simulink model "joystick_setup"  (R2018b)
settings: Solver=VariableStepAuto  StartTime=0.0  StopTime=30  RelTol=1e-3
libraries: joystick_lib x2, matlabinput_lib x1, aerolibanimutils x1
settings Model: Creator=Yannic  LastModifiedBy=jonas
settings DataIOCC: SaveOutput=off  SaveTime=off

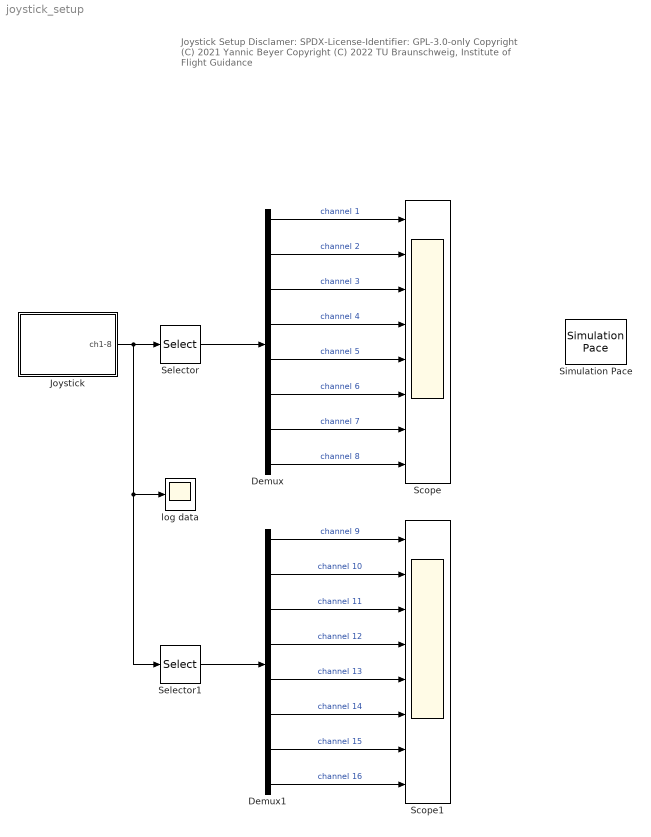
== system joystick_setup ==
  note: Joystick Setup
      |
      | Disclamer:
      | SPDX-License-Identifier: GPL-3.0-only
      |
      | Copyright (C) 2021 Yannic Beyer
      | Copyright (C) 2022 TU Braunschweig, Institute of Flight Guidance
  Demux : Demux  Outputs=8
  Demux1 : Demux  Outputs=8
  Joystick : Subsystem
  Scope : Scope  NumInputPorts=8
  Scope1 : Scope  NumInputPorts=8
  Selector : Selector  InputPortWidth=16  IndexOptions=Index vector (dialog)  Indices=1:8  OutputSizes=1
  Selector1 : Selector  InputPortWidth=16  IndexOptions=Index vector (dialog)  Indices=9:16  OutputSizes=1
  Simulation Pace : aerolibanimutils/Simulation Pace  SimulationPace=1  SleepMode=Auto  OutputPaceError=off  SampleTime=1/30
  log data : Scope
  wires:
  Demux/1 -> Scope/1  "channel 1"
  Demux/2 -> Scope/2  "channel 2"
  Demux/3 -> Scope/3  "channel 3"
  Demux/4 -> Scope/4  "channel 4"
  Demux/5 -> Scope/5  "channel 5"
  Demux/6 -> Scope/6  "channel 6"
  Demux/7 -> Scope/7  "channel 7"
  Demux/8 -> Scope/8  "channel 8"
  Selector/1 -> Demux/1
  Joystick/1(ch1-8) -> log data/1, Selector1/1, Selector/1
  Selector1/1 -> Demux1/1
  Demux1/8 -> Scope1/8  "channel 16"
  Demux1/7 -> Scope1/7  "channel 15"
  Demux1/2 -> Scope1/2  "channel 10"
  Demux1/6 -> Scope1/6  "channel 14"
  Demux1/4 -> Scope1/4  "channel 12"
  Demux1/5 -> Scope1/5  "channel 13"
  Demux1/3 -> Scope1/3  "channel 11"
  Demux1/1 -> Scope1/1  "channel 9"

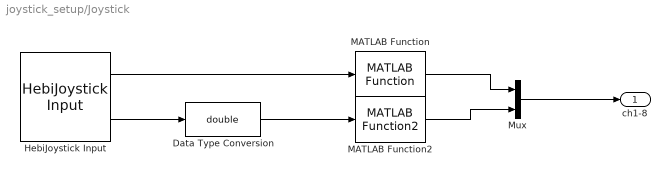
== system joystick_setup/Joystick ==
  Data Type Conversion : DataTypeConversion  OutDataTypeStr=double
  HebiJoystick Input : matlabinput_lib/HebiJoystick Input  joyid=1  forcefeed=off
      settings: SourceProductName=MatlabInput
  MATLAB Function : joystick_lib/Calibrated Joystick/MATLAB Function  SystemSampleTime=-1
      settings: SourceProductName=LADAC
  MATLAB Function2 : joystick_lib/Calibrated Joystick/MATLAB Function2  SystemSampleTime=-1
      settings: SourceProductName=LADAC
  Mux : Mux  Inputs=2
  ch1-8 : Outport
  wires:
  HebiJoystick Input/2 -> Data Type Conversion/1
  MATLAB Function/1 -> Mux/1
  HebiJoystick Input/1 -> MATLAB Function/1
  Data Type Conversion/1 -> MATLAB Function2/1
  Mux/1 -> ch1-8/1
  MATLAB Function2/1 -> Mux/2
